simulink model "sm_car_"  (R2026b)
settings: Solver=ode23t  StopTime=100  MaxStep=0.4  AbsTol=1e-3  EnableMultiTasking=on
PreLoadFcn:
  | % Due to usability issue in Repeating Sequence block
  | warning('off','Simulink:Masking:Invalid');
  | 
  | % Eliminate unnecessary warnings in inactive variants
  | % Warnings generated only if you click through inactive variant
  | warning('off','MATLAB:nonExistentField');
  | warning('off','Simulink:Parameters:BlkParamUndefined');
PostLoadFcn:
  | set_param([bdroot '/Vehicle'],'popup_trailer','Off')
  | warning('off','sm:sli:setup:compile:LocalSolverNotSupported')
  | %sm_car_config_maneuver(bdroot,'WOT Braking');
  | sm_car_config_vehicle(bdroot,'false');
  | sm_car_config_logging(bdroot);
InitFcn:
  | sm_car_config_camera;
  | Vehicle = sm_car_vehcfg_checkConfig(Vehicle);
  | sm_car_check_tire_model(bdroot);
StartFcn:
  | tic;
StopFcn:
  | Elapsed_Sim_Time = toc;
  | % disp(['Elapsed Sim Time = ' num2str(Elapsed_Sim_Time)]);
undefined symbols (not defined in the file or in its folder): acc_theta, accel_ramp_rate, Axle1D, AxleIn, Camera, Control, Driver, Init, Maneuver, Pedal, Scene, ShaftL1, ShaftL2, ShaftR1, ShaftR2, Visual, X, xy_data_car_side, Y, Z
libraries: sm_lib x290, fl_lib x171, nesl_utility x144, simulink x60, simulink_extras x14, sdl_lib x14, SimscapeFluids_lib x7, Damper_Element x4, Tire_1x2x x4, ee_lib x3, Scene_Utilities x3, sharedTrackingLibrary x2
(part 5 of 22)

== system sm_car_/Visualization/Data for Unreal ==
  VehBus : Inport
  DrvBus : Inport  Port=2
  Bus Selector : BusSelector  OutputSignals=aSteerWheel
  Bus Selector1 : BusSelector  OutputSignals=World.x,World.y,World.z  OutputAsBus=on
  Bus Selector2 : BusSelector  OutputSignals=World.aRoll,World.aPitch,World.aYaw  OutputAsBus=on
  Bus Selector5 : BusSelector  OutputSignals=Chassis.WhlL1.n,Chassis.WhlR1.n,Chassis.WhlL2.n,Chassis.WhlR2.n
  Bus Selector6 : BusSelector  OutputSignals=Chassis.WhlL1.aCamber,Chassis.WhlR1.aCamber,Chassis.WhlL2.aCamber,Chassis.WhlR2.aCamber
  Mux : Mux
  Mux1 : Mux
  xyz : Outport  VectorParamsAs1DForOutWhenUnconnected=off
  rpy : Outport  Port=2  VectorParamsAs1DForOutWhenUnconnected=off
  ws : Outport  Port=3  VectorParamsAs1DForOutWhenUnconnected=off
  aCamber : Outport  Port=4  VectorParamsAs1DForOutWhenUnconnected=off
  aSteerWheel : Outport  Port=5  VectorParamsAs1DForOutWhenUnconnected=off
  wires:
  Bus Selector/1 -> aSteerWheel/1  "<aSteerWheel>"
  Bus Selector6/4 -> Mux1/4  "<aCamber>"
  Bus Selector6/3 -> Mux1/3  "<aCamber>"
  Bus Selector6/2 -> Mux1/2  "<aCamber>"
  Mux/1 -> ws/1  "ws"
  Bus Selector2/1 -> rpy/1  "rpy"
  Bus Selector6/1 -> Mux1/1  "<aCamber>"
  Bus Selector5/1 -> Mux/1  "<n>"
  Bus Selector5/2 -> Mux/2  "<n>"
  Bus Selector5/4 -> Mux/4  "<n>"
  DrvBus/1 -> Bus Selector/1
  VehBus/1 -> Bus Selector1/1, Bus Selector2/1, Bus Selector5/1, Bus Selector6/1
  Mux1/1 -> aCamber/1  "aCamber"
  Bus Selector1/1 -> xyz/1  "xyz"
  Bus Selector5/3 -> Mux/3  "<n>"

== system sm_car_/Visualization/Mechanics Explorer Torque Bars ==
  CtrlBus : Inport
  RL 100 Percent Tick Offset : sm_lib/Frames and Transforms/Rigid Transform  RotationMethod=None  FollAlignAxisA=+X  BaseAlignAxisA=+Y  FollAlignAxisB=+Y  BaseAlignAxisB=+Z  RotationStandardAxis=+Z  RotationAngle=0  RotationAngleUnits=deg  RotationArbitraryAxis=[0 0 1]  RotationSequenceAxes=FollowerAxes  RotationSequence=XYX  RotationSequenceAngles=[0 0 0]  RotationSequenceAnglesUnits=deg  RotationMatrix=[1 0 0;0 1 0;0 0 1]  Quaternion=[1 0 0 0]  TranslationMethod=Cartesian  TranslationCartesianOffset=[0, 0, Visual.TorqueBars.travel]  TranslationCartesianOffsetUnits=m  TranslationStandardAxis=+Z  TranslationStandardOffset=0  TranslationStandardOffsetUnits=m  TranslationROffset=0  TranslationROffsetUnits=m  TranslationThetaOffset=0  TranslationThetaOffsetUnits=deg  TranslationZOffset=0  TranslationZOffsetUnits=m
  RL Bar Base : sm_lib/Frames and Transforms/Rigid Transform  RotationMethod=None  FollAlignAxisA=+X  BaseAlignAxisA=+Y  FollAlignAxisB=+Y  BaseAlignAxisB=+Z  RotationStandardAxis=+Z  RotationAngle=0  RotationAngleUnits=deg  RotationArbitraryAxis=[0 0 1]  RotationSequenceAxes=FollowerAxes  RotationSequence=XYX  RotationSequenceAngles=[0 0 0]  RotationSequenceAnglesUnits=deg  RotationMatrix=[1 0 0;0 1 0;0 0 1]  Quaternion=[1 0 0 0]  TranslationMethod=Cartesian  TranslationCartesianOffset=Vehicle.Chassis.Body.sAxle2.Value + [Vehicle.Chassis.SuspA2.Linkage.Upright.sWheelCentre.Value(1), abs(Vehicle.Chassis.SuspA2.Linkage.Upright.sWheelCentre.Value(2)) + Visual.TorqueBars.yOffset, Vehicle.Chassis.SuspA2.Linkage.Upright.sWheelCentre.Value(3) + Visual.TorqueBars.zOffset]  TranslationCartesianOffsetUnits=m  TranslationStandardAxis=+Z  TranslationStandardOffset=0  TranslationStandardOffsetUnits=m  TranslationROffset=0  TranslationROffsetUnits=m  TranslationThetaOffset=0  TranslationThetaOffsetUnits=deg  TranslationZOffset=0  TranslationZOffsetUnits=m
  RL Clip 0 100 : Saturate  UpperLimit=1  LowerLimit=0
  RL Demand Marker : sm_lib/Body Elements/Graphic  GraphicType=Marker  MarkerShape=Cube  MarkerSize=Visual.TorqueBars.markerSize +2  GraphicVisPropType=SimpleVisualProperties  GraphicDiffuseColor=Visual.TorqueBars.fill.clr  GraphicOpacity=Visual.TorqueBars.fill.opc*torque_bar_opacity_scale  GraphicSpecularColor=[0.5 0.5 0.5 1.0]  GraphicAmbientColor=[0.15 0.15 0.15 1.0]  GraphicEmissiveColor=[0.0 0.0 0.0 1.0]  GraphicShininess=75
  RL Demand Visual Memory : Memory
  RL Demand to Position : nesl_utility/Simulink-PS Converter  PhysicalDomain=network_engine_domain  SubClassName=ps_input  LeftPortType=input  RightPortType=output  PseudoPeriodic=off  Frequencies=[]  NoiseDistribution=none  NoiseParameters=[]  Unit=m  AffineConversion=off  FilteringAndDerivatives=filter  SimscapeFilterOrder=2  InputFilterTimeConstant=Visual.TorqueBars.filterTimeConstant  UdotUserProvided=0
  RL Full Tick : sm_lib/Body Elements/Graphic  GraphicType=Marker  MarkerShape=Cube  MarkerSize=Visual.TorqueBars.markerSize  GraphicVisPropType=SimpleVisualProperties  GraphicDiffuseColor=Visual.TorqueBars.tick.clr  GraphicOpacity=Visual.TorqueBars.tick.opc*torque_bar_opacity_scale  GraphicSpecularColor=[0.5 0.5 0.5 1.0]  GraphicAmbientColor=[0.15 0.15 0.15 1.0]  GraphicEmissiveColor=[0.0 0.0 0.0 1.0]  GraphicShininess=75
  RL Percent : Gain  Gain=1/max(Vehicle.Powertrain.Power.Motor.TorqueSpd.trq.Value)
  RL Toggle : Gain  Gain=torque_bar_enable
  RL Torque Slider : sm_lib/Joints/Prismatic Joint  JointMode=Normal  CompositeWrenchDir=FollowerOnBase  CompositeWrenchFrame=BaseFrame  SenseConstraintForce=off  SenseConstraintTorque=off  SenseTotalForce=off  SenseTotalTorque=off  PositionTargetSpecify=off  PositionTargetPriority=High  PositionTargetValue=0  PositionTargetValueUnits=m  VelocityTargetSpecify=off  VelocityTargetPriority=High  VelocityTargetValue=0  VelocityTargetValueUnits=m/s  EquilibriumPosition=0  EquilibriumPositionUnits=m  SpringStiffness=0  SpringStiffnessUnits=N/m  DampingCoefficient=0  DampingCoefficientUnits=N/(m/s)  LowerLimitSpecify=off  LowerLimitBound=-1  LowerLimitBoundUnits=m  LowerLimitStiffness=1e6  LowerLimitStiffnessUnits=N/m  LowerLimitDamping=1e3  LowerLimitDampingUnits=N/(m/s)  LowerLimitTransitionRegionWidth=1e-4  LowerLimitTransitionRegionWidthUnits=m  UpperLimitSpecify=off  UpperLimitBound=1  UpperLimitBoundUnits=m  UpperLimitStiffness=1e6  UpperLimitStiffnessUnits=N/m  UpperLimitDamping=1e3  UpperLimitDampingUnits=N/(m/s)  UpperLimitTransitionRegionWidth=1e-4  UpperLimitTransitionRegionWidthUnits=m  TorqueActuationMode=ComputedTorque  MotionActuationMode=InputMotion  SensePosition=off  SenseVelocity=off  SenseAcceleration=off  SenseTorqueForce=off  SenseLowerLimitTorqueForce=off  SenseUpperLimitTorqueForce=off
  RL Travel : Gain  Gain=Visual.TorqueBars.travel
  RL Zero Tick : sm_lib/Body Elements/Graphic  GraphicType=Marker  MarkerShape=Cube  MarkerSize=Visual.TorqueBars.markerSize  GraphicVisPropType=SimpleVisualProperties  GraphicDiffuseColor=Visual.TorqueBars.rail.clr  GraphicOpacity=Visual.TorqueBars.rail.opc*torque_bar_opacity_scale  GraphicSpecularColor=[0.5 0.5 0.5 1.0]  GraphicAmbientColor=[0.15 0.15 0.15 1.0]  GraphicEmissiveColor=[0.0 0.0 0.0 1.0]  GraphicShininess=75
  RR 100 Percent Tick Offset : sm_lib/Frames and Transforms/Rigid Transform  RotationMethod=None  FollAlignAxisA=+X  BaseAlignAxisA=+Y  FollAlignAxisB=+Y  BaseAlignAxisB=+Z  RotationStandardAxis=+Z  RotationAngle=0  RotationAngleUnits=deg  RotationArbitraryAxis=[0 0 1]  RotationSequenceAxes=FollowerAxes  RotationSequence=XYX  RotationSequenceAngles=[0 0 0]  RotationSequenceAnglesUnits=deg  RotationMatrix=[1 0 0;0 1 0;0 0 1]  Quaternion=[1 0 0 0]  TranslationMethod=Cartesian  TranslationCartesianOffset=[0, 0, Visual.TorqueBars.travel]  TranslationCartesianOffsetUnits=m  TranslationStandardAxis=+Z  TranslationStandardOffset=0  TranslationStandardOffsetUnits=m  TranslationROffset=0  TranslationROffsetUnits=m  TranslationThetaOffset=0  TranslationThetaOffsetUnits=deg  TranslationZOffset=0  TranslationZOffsetUnits=m
  RR Bar Base : sm_lib/Frames and Transforms/Rigid Transform  RotationMethod=None  FollAlignAxisA=+X  BaseAlignAxisA=+Y  FollAlignAxisB=+Y  BaseAlignAxisB=+Z  RotationStandardAxis=+Z  RotationAngle=0  RotationAngleUnits=deg  RotationArbitraryAxis=[0 0 1]  RotationSequenceAxes=FollowerAxes  RotationSequence=XYX  RotationSequenceAngles=[0 0 0]  RotationSequenceAnglesUnits=deg  RotationMatrix=[1 0 0;0 1 0;0 0 1]  Quaternion=[1 0 0 0]  TranslationMethod=Cartesian  TranslationCartesianOffset=Vehicle.Chassis.Body.sAxle2.Value + [Vehicle.Chassis.SuspA2.Linkage.Upright.sWheelCentre.Value(1), -(abs(Vehicle.Chassis.SuspA2.Linkage.Upright.sWheelCentre.Value(2)) + Visual.TorqueBars.yOffset), Vehicle.Chassis.SuspA2.Linkage.Upright.sWheelCentre.Value(3) + Visual.TorqueBars.zOffset]  TranslationCartesianOffsetUnits=m  TranslationStandardAxis=+Z  TranslationStandardOffset=0  TranslationStandardOffsetUnits=m  TranslationROffset=0  TranslationROffsetUnits=m  TranslationThetaOffset=0  TranslationThetaOffsetUnits=deg  TranslationZOffset=0  TranslationZOffsetUnits=m
  RR Clip 0 100 : Saturate  UpperLimit=1  LowerLimit=0
  RR Demand Marker : sm_lib/Body Elements/Graphic  GraphicType=Marker  MarkerShape=Cube  MarkerSize=Visual.TorqueBars.markerSize +2  GraphicVisPropType=SimpleVisualProperties  GraphicDiffuseColor=Visual.TorqueBars.fill.clr  GraphicOpacity=Visual.TorqueBars.fill.opc*torque_bar_opacity_scale  GraphicSpecularColor=[0.5 0.5 0.5 1.0]  GraphicAmbientColor=[0.15 0.15 0.15 1.0]  GraphicEmissiveColor=[0.0 0.0 0.0 1.0]  GraphicShininess=75
  RR Demand Visual Memory : Memory
  RR Demand to Position : nesl_utility/Simulink-PS Converter  PhysicalDomain=network_engine_domain  SubClassName=ps_input  LeftPortType=input  RightPortType=output  PseudoPeriodic=off  Frequencies=[]  NoiseDistribution=none  NoiseParameters=[]  Unit=m  AffineConversion=off  FilteringAndDerivatives=filter  SimscapeFilterOrder=2  InputFilterTimeConstant=Visual.TorqueBars.filterTimeConstant  UdotUserProvided=0
  RR Full Tick : sm_lib/Body Elements/Graphic  GraphicType=Marker  MarkerShape=Cube  MarkerSize=Visual.TorqueBars.markerSize  GraphicVisPropType=SimpleVisualProperties  GraphicDiffuseColor=Visual.TorqueBars.tick.clr  GraphicOpacity=Visual.TorqueBars.tick.opc*torque_bar_opacity_scale  GraphicSpecularColor=[0.5 0.5 0.5 1.0]  GraphicAmbientColor=[0.15 0.15 0.15 1.0]  GraphicEmissiveColor=[0.0 0.0 0.0 1.0]  GraphicShininess=75
  RR Percent : Gain  Gain=1/max(Vehicle.Powertrain.Power.Motor.TorqueSpd.trq.Value)
  RR Toggle : Gain  Gain=torque_bar_enable
  RR Torque Slider : sm_lib/Joints/Prismatic Joint  JointMode=Normal  CompositeWrenchDir=FollowerOnBase  CompositeWrenchFrame=BaseFrame  SenseConstraintForce=off  SenseConstraintTorque=off  SenseTotalForce=off  SenseTotalTorque=off  PositionTargetSpecify=off  PositionTargetPriority=High  PositionTargetValue=0  PositionTargetValueUnits=m  VelocityTargetSpecify=off  VelocityTargetPriority=High  VelocityTargetValue=0  VelocityTargetValueUnits=m/s  EquilibriumPosition=0  EquilibriumPositionUnits=m  SpringStiffness=0  SpringStiffnessUnits=N/m  DampingCoefficient=0  DampingCoefficientUnits=N/(m/s)  LowerLimitSpecify=off  LowerLimitBound=-1  LowerLimitBoundUnits=m  LowerLimitStiffness=1e6  LowerLimitStiffnessUnits=N/m  LowerLimitDamping=1e3  LowerLimitDampingUnits=N/(m/s)  LowerLimitTransitionRegionWidth=1e-4  LowerLimitTransitionRegionWidthUnits=m  UpperLimitSpecify=off  UpperLimitBound=1  UpperLimitBoundUnits=m  UpperLimitStiffness=1e6  UpperLimitStiffnessUnits=N/m  UpperLimitDamping=1e3  UpperLimitDampingUnits=N/(m/s)  UpperLimitTransitionRegionWidth=1e-4  UpperLimitTransitionRegionWidthUnits=m  TorqueActuationMode=ComputedTorque  MotionActuationMode=InputMotion  SensePosition=off  SenseVelocity=off  SenseAcceleration=off  SenseTorqueForce=off  SenseLowerLimitTorqueForce=off  SenseUpperLimitTorqueForce=off
  RR Travel : Gain  Gain=Visual.TorqueBars.travel
  RR Zero Tick : sm_lib/Body Elements/Graphic  GraphicType=Marker  MarkerShape=Cube  MarkerSize=Visual.TorqueBars.markerSize  GraphicVisPropType=SimpleVisualProperties  GraphicDiffuseColor=Visual.TorqueBars.rail.clr  GraphicOpacity=Visual.TorqueBars.rail.opc*torque_bar_opacity_scale  GraphicSpecularColor=[0.5 0.5 0.5 1.0]  GraphicAmbientColor=[0.15 0.15 0.15 1.0]  GraphicEmissiveColor=[0.0 0.0 0.0 1.0]  GraphicShininess=75
  Rear Motor Demands : BusSelector  OutputSignals=Power.MMotorL2Demand,Power.MMotorR2Demand
  Vehicle Frame : PMIOPort  Side=Left
  wires:
  RL Travel/1 -> RL Demand to Position/1
  RL Toggle/1 -> RL Travel/1
  RR Percent/1 -> RR Clip 0 100/1
  RR Toggle/1 -> RR Travel/1
  RL Clip 0 100/1 -> RL Toggle/1
  RR Travel/1 -> RR Demand to Position/1
  CtrlBus/1 -> Rear Motor Demands/1
  RL Percent/1 -> RL Clip 0 100/1
  RR Clip 0 100/1 -> RR Toggle/1
  Rear Motor Demands/1 -> RL Demand Visual Memory/1  "<MMotorL2Demand>"
  RL Demand Visual Memory/1 -> RL Percent/1  "MMotorL2Demand"
  Rear Motor Demands/2 -> RR Demand Visual Memory/1  "<MMotorR2Demand>"
  RR Demand Visual Memory/1 -> RR Percent/1  "MMotorR2Demand"
  connections:
  RR 100 Percent Tick Offset/RConn1 -- RR Full Tick/RConn1
  RR Torque Slider/RConn1 -- RR Demand Marker/RConn1
  RR Bar Base/RConn1 -- RR 100 Percent Tick Offset/LConn1 -- RR Torque Slider/LConn1 -- RR Zero Tick/RConn1
  RL Demand to Position/RConn1 -- RL Torque Slider/LConn2
  Vehicle Frame/RConn1 -- RR Bar Base/LConn1 -- RL Bar Base/LConn1
  RL Torque Slider/RConn1 -- RL Demand Marker/RConn1
  RL 100 Percent Tick Offset/RConn1 -- RL Full Tick/RConn1
  RL Zero Tick/RConn1 -- RL Torque Slider/LConn1 -- RL Bar Base/RConn1 -- RL 100 Percent Tick Offset/LConn1
  RR Demand to Position/RConn1 -- RR Torque Slider/LConn2

== system sm_car_/Visualization/Unreal ==
  "xyz " : Inport
  "rpy " : Inport  Port=2
  "ws " : Inport  Port=3
  "aCamber " : Inport  Port=4
  "aSteerWheel " : Inport  Port=5
  Animation Off : Subsystem  VariantControl=Off

== system sm_car_/World/Mechanism Configuration ==
  Constant Gravity : Subsystem  VariantControl=ConstantGravity
  Variable GravityXY : Subsystem  VariantControl=VariableGravityXY
  C : PMIOPort  Side=Right

== system sm_car_/World/Scene ==
  CRG Balkans : sm_car_scene_crg_balkans/CRG Balkans  VariantControl=CRG_Balkans  geometry=Scene.CRG_Balkans.Geometry
  CRG Balkans End : sm_car_scene_crg_balkans_end/CRG Balkans End  VariantControl=CRG_Balkans_End  geometry=Scene.CRG_Balkans_End.Geometry
  CRG Balkans End F : sm_car_scene_crg_balkans_end_f/CRG Balkans End F  VariantControl=CRG_Balkans_End_F  geometry=Scene.CRG_Balkans_End_F.Geometry
  CRG Balkans F : sm_car_scene_crg_balkans_f/CRG Balkans F  VariantControl=CRG_Balkans_F  geometry=Scene.CRG_Balkans_F.Geometry
  CRG Dej Wide : sm_car_scene_crg_dej_wide/CRG Dej Wide  VariantControl=CRG_Dej_Wide  geometry=Scene.CRG_Dej_Wide.Geometry
  CRG Dej Wide F : sm_car_scene_crg_dej_wide_f/CRG Dej Wide F  VariantControl=CRG_Dej_Wide_F  geometry=Scene.CRG_Dej_Wide_F.Geometry
  CRG Germania : sm_car_scene_crg_germania/CRG Germania  VariantControl=CRG_Germania  geometry=Scene.CRG_Germania.Geometry
  CRG Germania F : sm_car_scene_crg_germania_f/CRG Germania F  VariantControl=CRG_Germania_F  geometry=Scene.CRG_Germania_F.Geometry
  CRG Hockenheim : Subsystem  VariantControl=CRG_Hockenheim  mask{geometry=Scene.CRG_Hockenheim.Geometry}
      mask prompts: geometry "Geometry (structure)"
  CRG Hockenheim F : Subsystem  VariantControl=CRG_Hockenheim_F  mask{geometry=Scene.CRG_Hockenheim_F.Geometry}
      mask prompts: geometry "Geometry (structure)"
  Double Lane Change : Subsystem  VariantControl=Double_Lane_Change  mask{road=Scene.Double_Lane_Change.Road, dashes=Scene.Double_Lane_Change.Dashes, cones=Scene.Double_Lane_Change.Cones}
      mask prompts: road "Road (structure)"; dashes "Dashes (structure)"; cones "Cones (structure)"
  Plane Grid : Subsystem  VariantControl=Plane_Grid  mask{plane=Scene.Plane_Grid.Plane, grid=Scene.Plane_Grid.Grid}
      mask prompts: plane "Ground Plane (structure)"; grid "Grid (structure)"
  Skidpad : Subsystem  VariantControl=Skidpad  mask{circ_in=Scene.Skidpad.Circle_Inner, circ_out=Scene.Skidpad.Circle_Outer, plane=Scene.Skidpad.Plane}
      mask prompts: circ_in "Circle Inner (structure)"; circ_out "Circle Outer (structure)"; plane "Plane (structure)"
  Slalom : sm_car_scene_slalom/Slalom  VariantControl=Slalom  road=Scene.Slalom.Road  dashes=Scene.Slalom.Dashes  cones=Scene.Slalom.Cones  vehTraj=Maneuver.Trajectory
  W : PMIOPort  Side=Left
  Obs : Outport  VectorParamsAs1DForOutWhenUnconnected=off

== system sm_car_/Camera Frames/Dolly Camera/Off ==
  W : PMIOPort  Side=Left
  R : PMIOPort  Port=2  Side=Right
  connections:
  R/RConn1 -- W/RConn1

== system sm_car_/Controller/Default/Brake Control ==
  "rBrakePedal " : Inport
  "VehBus " : Inport  Port=2
  Pedal : Subsystem  VariantControl=Pedal
  " Brakes" : Outport  VectorParamsAs1DForOutWhenUnconnected=off

== system sm_car_/Controller/Default/Driveline Control ==
  Bus Creator : BusCreator  Inputs=1
  Constant : Constant  Value=0
  Driveline : Outport  VectorParamsAs1DForOutWhenUnconnected=off
  wires:
  Bus Creator/1 -> Driveline/1  "Driveline"
  Constant/1 -> Bus Creator/1  "placeholder"

== system sm_car_/Controller/Default/Power Control ==
  note: For 4 Motor Powertrain only
  note: For 2 Motor Powertrain only
  rAccelPedal : Inport
  VehBus : Inport  Port=2
  StatesEst : Inport  Port=3
  1-D Lookup Table : Lookup_n-D  NumberOfTableDimensions=1  BreakpointsForDimension1=[0;400;4600]  Table=[0;3;8]  InternalRulePriority=Speed  RndMeth=Simplest
  1-D Lookup Table1 : Lookup_n-D  NumberOfTableDimensions=1  BreakpointsForDimension1=[-1;-0.20000000000000001;-0.10000000000000001;0;0.10000000000000001;0.20000000000000001;1]  Table=[0;0;1;1;1;0;0]  InternalRulePriority=Speed  RndMeth=Simplest
  1-D Lookup Table2 : Lookup_n-D  NumberOfTableDimensions=1  BreakpointsForDimension1=[0;400;4600]  Table=[0;3;8]  InternalRulePriority=Speed  RndMeth=Simplest
  Add : Sum
  Add1 : Sum
  Bus Creator : BusCreator  Inputs=7
  Bus Selector : BusSelector  OutputSignals=Power.MotorL2.w,Power.MotorR2.w
  Constant : Constant  Value=trq_ratio_front
  Constant1 : Constant  Value=0
  Constant2 : Constant
  Gain : Gain  Gain=max(Vehicle.Powertrain.Power.Motor.TorqueSpd.trq.Value)
  Gain1 : Gain  Gain=-1
  Gain2 : Gain  Gain=-1
  Gain3 : Gain  Gain=0.5
  Gain4 : Gain  Gain=0.5
  Product{,1..3} (4 alike) : Product
  Rate Limiter : RateLimiter  RisingSlewLimit=trq_rate_up  FallingSlewLimit=trq_rate_down  SampleTimeMode=inherited
  Terminator1 : Terminator
  Power : Outport  VectorParamsAs1DForOutWhenUnconnected=off
  wires:
  Bus Creator/1 -> Power/1  "Power"
  Product1/1 -> Add1/1, Add/1, Bus Creator/4  "MMotorA2Demand"
  Gain/1 -> 1-D Lookup Table1/1, Rate Limiter/1
  Product/1 -> Gain4/1, Gain3/1, Bus Creator/1  "MMotorA1Demand"
  rAccelPedal/1 -> Gain/1
  VehBus/1 -> Bus Selector/1
  Constant1/1 -> Bus Creator/7  "MRegenBrakeLimit"
  Rate Limiter/1 -> Product1/1, Product/2
  Constant/1 -> Product/1
  Constant2/1 -> Product1/2
  Add/1 -> Bus Creator/5  "MMotorL2Demand"
  Add1/1 -> Bus Creator/6  "MMotorR2Demand"
  Gain3/1 -> Bus Creator/2  "MMotorL1Demand"
  Gain4/1 -> Bus Creator/3  "MMotorR1Demand"
  StatesEst/1 -> Terminator1/1
  Bus Selector/1 -> 1-D Lookup Table/1  "<w>"
  Bus Selector/2 -> 1-D Lookup Table2/1  "<w>"
  1-D Lookup Table/1 -> Gain1/1
  1-D Lookup Table1/1 -> Product3/1, Product2/1
  1-D Lookup Table2/1 -> Gain2/1
  Product2/1 -> Add/2
  Product3/1 -> Add1/2
  Gain1/1 -> Product2/2
  Gain2/1 -> Product3/2

== system sm_car_/Controller/Default/Spring Damper ==
  Bus Creator : BusCreator  Inputs=4
  Bus Creator1 : BusCreator  Inputs=4
  Constant : Constant  Value=[0 0 0 0]
  Constant1 : Constant  Value=[0 0 0 0]
  Demux : Demux
  Demux1 : Demux
  Damper : Outport  VectorParamsAs1DForOutWhenUnconnected=off
  Spring : Outport  Port=2  VectorParamsAs1DForOutWhenUnconnected=off
  wires:
  Constant/1 -> Demux/1
  Demux/3 -> Bus Creator/3  "L2"
  Demux/4 -> Bus Creator/4  "R2"
  Demux/1 -> Bus Creator/1  "L1"
  Demux/2 -> Bus Creator/2  "R1"
  Demux1/2 -> Bus Creator1/2  "R1"
  Demux1/1 -> Bus Creator1/1  "L1"
  Demux1/4 -> Bus Creator1/4  "R2"
  Demux1/3 -> Bus Creator1/3  "L2"
  Constant1/1 -> Demux1/1
  Bus Creator1/1 -> Damper/1  "Damper"
  Bus Creator/1 -> Spring/1  "Spring"

== system sm_car_/Controller/Default/State Estimation ==
  aSteerWheel : Inport
  VehBus : Inport  Port=2
  Bus Creator : BusCreator  Inputs=5
  Bus Selector : BusSelector  OutputSignals=World.vx,World.vy,World.vz,Chassis.Body.CG.nYaw,Chassis.Body.CG.gx,Chassis.Body.CG.gy,Chassis.SuspA1.LinkageL.Upright.Upright.w,Chassis.SuspA1.LinkageR.Upright.Upright.w,Chassis.SuspA2.LinkageL.Upright.Upright.w,Chassis.SuspA2.LinkageR.Upright.Upright.w
  Data Type Conversion : DataTypeConversion  OutDataTypeStr=double  SaturateOnIntegerOverflow=off  RndMeth=Floor
  Data Type Conversion1 : DataTypeConversion  OutDataTypeStr=double  SaturateOnIntegerOverflow=off  RndMeth=Floor
  Demux : Demux  Outputs=5
  Rate Transition1 : RateTransition  Deterministic=off  OutPortSampleTime=0.003
  Rate Transition2 : RateTransition  Deterministic=off  OutPortSampleTime=0.003
  Rate Transition4 : RateTransition  Deterministic=off
  Sensor Noise Simulation : Subsystem
  UKF : Subsystem
  StateEst : Outport
  Out Bus Element : Outport  Port=2  PortName=Meas  Element=Meas
  Out Bus Element1 : Outport  Port=2  PortName=Meas  Element=Input
  Out Bus Element2 : Outport  Port=2  PortName=Meas  Element=State
  wires:
  VehBus/1 -> Bus Selector/1
  Bus Selector/1 -> Sensor Noise Simulation/1(<vx>)  "<vx>"
  Bus Selector/2 -> Sensor Noise Simulation/2(<vy>)  "<vy>"
  Bus Selector/4 -> Sensor Noise Simulation/4(<nYaw>)  "<nYaw>"
  Bus Selector/5 -> Sensor Noise Simulation/5(<gx>)  "<gx>"
  Bus Selector/6 -> Sensor Noise Simulation/6(<gy>)  "<gy>"
  Bus Selector/7 -> Sensor Noise Simulation/7(<w_fl>)  "<w>"
  Bus Selector/8 -> Sensor Noise Simulation/8(<w_fr>)  "<w>"
  Bus Selector/9 -> Sensor Noise Simulation/9(<w_rl>)  "<w>"
  Bus Selector/10 -> Sensor Noise Simulation/10(<w_rr>)  "<w>"
  aSteerWheel/1 -> Sensor Noise Simulation/11(delta)  "delta"
  Sensor Noise Simulation/2(Meas) -> Rate Transition2/1, Out Bus Element/1  "Measument"
  Sensor Noise Simulation/1(Inputs) -> Data Type Conversion1/1, Rate Transition1/1  "Input"
  Data Type Conversion/1 -> Demux/1
  Bus Creator/1 -> Out Bus Element2/1, StateEst/1  "UKF"
  Demux/1 -> Bus Creator/1  "v_x"
  Demux/2 -> Bus Creator/2  "v_y"
  Demux/3 -> Bus Creator/3  "phi_dot"
  Demux/4 -> Bus Creator/4  "a_x"
  Demux/5 -> Bus Creator/5  "a_y"
  Rate Transition1/1 -> UKF/1(StateTransitionFcnInputs)
  Rate Transition2/1 -> UKF/2(y1)
  UKF/1(xhat) -> Data Type Conversion/1
  Data Type Conversion1/1 -> Rate Transition4/1
  Rate Transition4/1 -> Out Bus Element1/1
  Bus Selector/3 -> Sensor Noise Simulation/3(<vz>)  "<vz>"

== system sm_car_/Controller/Default/Susp ==
  aSteerWheel : Inport
  vx : Inport  Port=2
  1-D Lookup Table : Lookup_n-D  NumberOfTableDimensions=1  BreakpointsForDimension1=Steer.Gain.vVehicle.Value  Table=Steer.Gain.n.Value  InterpMethod=Linear Lagrange  InternalRulePriority=Speed  RndMeth=Simplest
  Bus Creator{1..4} (4 alike) : BusCreator  Inputs=1
  Gain : Gain  Gain=3.6
  Product : Product
  Saturation : Saturate  UpperLimit=Steer.Limits.aUpper.Value  LowerLimit=Steer.Limits.aLower.Value  LinearizeAsGain=off  ZeroCross=off
  Transfer Fcn (with initial states) : simulink_extras/Additional Linear/Transfer Fcn (with initial states)  N=[1]  D="[1/Steer.fActuatorCutoff.Value  1]"  X0=-1
  SuspA1 : Outport  VectorParamsAs1DForOutWhenUnconnected=off
  SuspA2 : Outport  Port=2  VectorParamsAs1DForOutWhenUnconnected=off
  wires:
  Bus Creator4/1 -> Bus Creator1/1  "Steer"
  Bus Creator2/1 -> Bus Creator3/1  "Steer"
  Bus Creator3/1 -> SuspA2/1  "SuspA2"
  Bus Creator1/1 -> SuspA1/1  "SuspA1"
  aSteerWheel/1 -> Product/1, Bus Creator4/1  "aSteerWheel"
  Saturation/1 -> Bus Creator2/1  "aSteerWheel"
  vx/1 -> Gain/1
  Transfer Fcn (with initial states)/1 -> Product/2
  Product/1 -> Saturation/1
  Gain/1 -> 1-D Lookup Table/1
  1-D Lookup Table/1 -> Transfer Fcn (with initial states)/1

== system sm_car_/Controller/FeedF_Ctrl/Brake Control ==
  "rBrakePedal " : Inport
  "VehBus " : Inport  Port=2
  Pedal : Subsystem  VariantControl=Pedal
  " Brakes" : Outport  VectorParamsAs1DForOutWhenUnconnected=off

== system sm_car_/Controller/FeedF_Ctrl/Driveline Control ==
  Bus Creator : BusCreator  Inputs=1
  Constant : Constant  Value=0
  Driveline : Outport  VectorParamsAs1DForOutWhenUnconnected=off
  wires:
  Constant/1 -> Bus Creator/1  "placeholder"
  Bus Creator/1 -> Driveline/1  "Driveline"

== system sm_car_/Controller/FeedF_Ctrl/Power Control ==
  rAccelPedal : Inport
  VehBus : Inport  Port=2
  aSteerWheel : Inport  Port=3
  Bias : Bias  Bias=512  SaturateOnIntegerOverflow=off
  Bus Creator : BusCreator  Inputs=2
  Bus Selector : BusSelector  OutputSignals=Power.MotorL2.w,Power.MotorR2.w
  Gain : Gain  Gain=max(Control.MotorTrq)
  Gain1 : Gain  Gain=max(Control.MotorTrq)
  Gain3 : Gain  Gain=511/154
  Radians to Degrees : simulink_extras/Transformations/Radians to Degrees
  Subsystem Reference : Subsystem  ReferencedSubsystem=FeedForward  rwheel=Control.WheelRad  L=Control.Wheelbase  StrWhlRatio=Control.StrWheelRatio  Izz=Control.Izz  tr=Control.RearTrack  Gr=Control.GearRatio  MotorT=Control.MotorTrq  MotorW=Control.MotorW  Tf=0.005  Tmax=max(Control.MotorTrq)  Ku=Control.UndersteerGradient
  Power : Outport  VectorParamsAs1DForOutWhenUnconnected=off
  wires:
  Bias/1 -> Subsystem Reference/1
  Gain3/1 -> Bias/1
  Radians to Degrees/1 -> Gain3/1
  Gain1/1 -> Bus Creator/2  "MMotorR2Demand"
  Gain/1 -> Bus Creator/1  "MMotorL2Demand"
  Subsystem Reference/2 -> Gain1/1  "MMotorR2Demand"
  Subsystem Reference/1 -> Gain/1  "MMotorL2Demand"
  Bus Creator/1 -> Power/1
  rAccelPedal/1 -> Subsystem Reference/4  "Throttle[~]"
  aSteerWheel/1 -> Radians to Degrees/1  "Throttle[~]"
  VehBus/1 -> Bus Selector/1
  Bus Selector/1 -> Subsystem Reference/2  "<w>"
  Bus Selector/2 -> Subsystem Reference/3  "<w>"

== system sm_car_/Controller/FeedF_Ctrl/Spring Damper ==
  Bus Creator : BusCreator  Inputs=4
  Bus Creator1 : BusCreator  Inputs=4
  Constant : Constant  Value=[0 0 0 0]
  Constant1 : Constant  Value=[0 0 0 0]
  Demux : Demux
  Demux1 : Demux
  Damper : Outport  VectorParamsAs1DForOutWhenUnconnected=off
  Spring : Outport  Port=2  VectorParamsAs1DForOutWhenUnconnected=off
  wires:
  Bus Creator/1 -> Spring/1  "Spring"
  Bus Creator1/1 -> Damper/1  "Damper"
  Constant1/1 -> Demux1/1
  Demux1/3 -> Bus Creator1/3  "L2"
  Demux1/4 -> Bus Creator1/4  "R2"
  Demux1/1 -> Bus Creator1/1  "L1"
  Demux1/2 -> Bus Creator1/2  "R1"
  Demux/2 -> Bus Creator/2  "R1"
  Demux/1 -> Bus Creator/1  "L1"
  Demux/4 -> Bus Creator/4  "R2"
  Demux/3 -> Bus Creator/3  "L2"
  Constant/1 -> Demux/1

== system sm_car_/Controller/FeedF_Ctrl/Susp ==
  aSteerWheel : Inport
  vx : Inport  Port=2
  1-D Lookup Table : Lookup_n-D  NumberOfTableDimensions=1  BreakpointsForDimension1=Steer.Gain.vVehicle.Value  Table=Steer.Gain.n.Value  InterpMethod=Linear Lagrange  InternalRulePriority=Speed  RndMeth=Simplest
  Bus Creator{1..4} (4 alike) : BusCreator  Inputs=1
  Gain : Gain  Gain=3.6
  Product : Product
  Saturation : Saturate  UpperLimit=Steer.Limits.aUpper.Value  LowerLimit=Steer.Limits.aLower.Value  LinearizeAsGain=off  ZeroCross=off
  Transfer Fcn (with initial states) : simulink_extras/Additional Linear/Transfer Fcn (with initial states)  N=[1]  D="[1/Steer.fActuatorCutoff.Value  1]"  X0=-1
  SuspA1 : Outport  VectorParamsAs1DForOutWhenUnconnected=off
  SuspA2 : Outport  Port=2  VectorParamsAs1DForOutWhenUnconnected=off
  wires:
  1-D Lookup Table/1 -> Transfer Fcn (with initial states)/1
  Gain/1 -> 1-D Lookup Table/1
  Product/1 -> Saturation/1
  Transfer Fcn (with initial states)/1 -> Product/2
  vx/1 -> Gain/1
  Saturation/1 -> Bus Creator2/1  "aSteerWheel"
  aSteerWheel/1 -> Bus Creator4/1, Product/1  "aSteerWheel"
  Bus Creator1/1 -> SuspA1/1  "SuspA1"
  Bus Creator3/1 -> SuspA2/1  "SuspA2"
  Bus Creator2/1 -> Bus Creator3/1  "Steer"
  Bus Creator4/1 -> Bus Creator1/1  "Steer"

== system sm_car_/Controller/NoIMU/Brake Control ==
  "rBrakePedal " : Inport
  "VehBus " : Inport  Port=2
  Pedal : Subsystem  VariantControl=Pedal
  " Brakes" : Outport  VectorParamsAs1DForOutWhenUnconnected=off

== system sm_car_/Controller/NoIMU/Driveline Control ==
  Bus Creator : BusCreator  Inputs=1
  Constant : Constant  Value=0
  Driveline : Outport  VectorParamsAs1DForOutWhenUnconnected=off
  wires:
  Constant/1 -> Bus Creator/1  "placeholder"
  Bus Creator/1 -> Driveline/1  "Driveline"

== system sm_car_/Controller/NoIMU/Power Control ==
  rAccelPedal : Inport
  VehBus : Inport  Port=2
  Add1 : Sum
  Bus Creator : BusCreator  Inputs=2
  Bus Creator2 : BusCreator  Inputs=2
  Bus Selector : BusSelector  OutputSignals=Power.Battery.v,Power.MotorL2.i,Power.MotorR2.i
  Constant : Constant
  Current-Torque : Subsystem
  Delay : Delay  DelayLength=1  InputProcessing=Columns as channels (frame based)
  Fuzzy Logic Controller : fuzblock/Fuzzy Logic  Controller  FIS=fis  OutputSampleNumber=101  DataType=double  UseLookupTable=off  NumBreakpoints=10  FuzzifiedInputs=off  RuleFiringStrengths=off  RuleOutputs=off  AggregatedOutputs=off  SimulateUsing=Interpreted execution  OutOfRangeInputValueMessage=warning  NoRuleFiredMessage=warning  EmptyOutputFuzzySetMessage=warning
  Product : Product
  Product1 : Product
  Product2 : Product  Inputs=3
  Saturation : Saturate  UpperLimit=1  LowerLimit=0
  Slip Control : Subsystem  Commented=on
  Subtract : Sum  Inputs=+-
  Sum : Sum  Inputs=|+-
  Tmax : Gain  Gain=1/Tmax/2
  max torque : Constant  Value=Tmax
  Power : Outport  VectorParamsAs1DForOutWhenUnconnected=off
  wires:
  VehBus/1 -> Slip Control/1(VehBus), Bus Selector/1
  Bus Creator/1 -> Power/1  "Power"
  rAccelPedal/1 -> Sum/1, Product2/1  "Throttle[~]"
  Bus Selector/1 -> Current-Torque/1(V)  "<v>"
  Bus Selector/2 -> Current-Torque/2(Il)  "<i>"
  Bus Selector/3 -> Current-Torque/3(Ir)  "<i>"
  Fuzzy Logic Controller/1 -> Add1/2
  Current-Torque/1(Out1) -> Tmax/1  "Treal[Nm]"
  Bus Creator2/1 -> ?
  Product2/1 -> Product/1, Product1/1  "MDemand[Nm]"
  Tmax/1 -> Saturation/1
  Saturation/1 -> Sum/2  "Treal[%]"
  max torque/1 -> Product2/3
  Add1/1 -> Product2/2
  Sum/1 -> Delay/1, Subtract/1, Bus Creator2/1
  Delay/1 -> Subtract/2
  Subtract/1 -> Bus Creator2/2
  Constant/1 -> Add1/1
  Product/1 -> Bus Creator/2  "MMotorR2Demand"
  Product1/1 -> Bus Creator/1  "MMotorL2Demand"
  Slip Control/1(Out1) -> Product1/2
  Slip Control/2(Out2) -> Product/2

== system sm_car_/Controller/NoIMU/Spring Damper ==
  Bus Creator : BusCreator  Inputs=4
  Bus Creator1 : BusCreator  Inputs=4
  Constant : Constant  Value=[0 0 0 0]
  Constant1 : Constant  Value=[0 0 0 0]
  Demux : Demux
  Demux1 : Demux
  Damper : Outport  VectorParamsAs1DForOutWhenUnconnected=off
  Spring : Outport  Port=2  VectorParamsAs1DForOutWhenUnconnected=off
  wires:
  Bus Creator/1 -> Spring/1  "Spring"
  Bus Creator1/1 -> Damper/1  "Damper"
  Constant1/1 -> Demux1/1
  Demux1/3 -> Bus Creator1/3  "L2"
  Demux1/4 -> Bus Creator1/4  "R2"
  Demux1/1 -> Bus Creator1/1  "L1"
  Demux1/2 -> Bus Creator1/2  "R1"
  Demux/2 -> Bus Creator/2  "R1"
  Demux/1 -> Bus Creator/1  "L1"
  Demux/4 -> Bus Creator/4  "R2"
  Demux/3 -> Bus Creator/3  "L2"
  Constant/1 -> Demux/1

== system sm_car_/Controller/NoIMU/Susp ==
  aSteerWheel : Inport
  vx : Inport  Port=2
  1-D Lookup Table : Lookup_n-D  NumberOfTableDimensions=1  BreakpointsForDimension1=Steer.Gain.vVehicle.Value  Table=Steer.Gain.n.Value  InterpMethod=Linear Lagrange  InternalRulePriority=Speed  RndMeth=Simplest
  Bus Creator{1..4} (4 alike) : BusCreator  Inputs=1
  Gain : Gain  Gain=3.6
  Product : Product
  Saturation : Saturate  UpperLimit=Steer.Limits.aUpper.Value  LowerLimit=Steer.Limits.aLower.Value  LinearizeAsGain=off  ZeroCross=off
  Transfer Fcn (with initial states) : simulink_extras/Additional Linear/Transfer Fcn (with initial states)  N=[1]  D="[1/Steer.fActuatorCutoff.Value  1]"  X0=-1
  SuspA1 : Outport  VectorParamsAs1DForOutWhenUnconnected=off
  SuspA2 : Outport  Port=2  VectorParamsAs1DForOutWhenUnconnected=off
  wires:
  1-D Lookup Table/1 -> Transfer Fcn (with initial states)/1
  Gain/1 -> 1-D Lookup Table/1
  Product/1 -> Saturation/1
  Transfer Fcn (with initial states)/1 -> Product/2
  vx/1 -> Gain/1
  Saturation/1 -> Bus Creator2/1  "aSteerWheel"
  aSteerWheel/1 -> Bus Creator4/1, Product/1  "aSteerWheel"
  Bus Creator1/1 -> SuspA1/1  "SuspA1"
  Bus Creator3/1 -> SuspA2/1  "SuspA2"
  Bus Creator2/1 -> Bus Creator3/1  "Steer"
  Bus Creator4/1 -> Bus Creator1/1  "Steer"

== system sm_car_/Controller/Slip_Ctrl/Brake Control ==
  "rBrakePedal " : Inport
  "VehBus " : Inport  Port=2
  Pedal : Subsystem  VariantControl=Pedal
  " Brakes" : Outport  VectorParamsAs1DForOutWhenUnconnected=off

== system sm_car_/Controller/Slip_Ctrl/Driveline Control ==
  Bus Creator : BusCreator  Inputs=1
  Constant : Constant  Value=0
  Driveline : Outport  VectorParamsAs1DForOutWhenUnconnected=off
  wires:
  Constant/1 -> Bus Creator/1  "placeholder"
  Bus Creator/1 -> Driveline/1  "Driveline"

== system sm_car_/Controller/Slip_Ctrl/Power Control ==
  rAccelPedal : Inport
  VehBus : Inport  Port=2
  Bus Creator : BusCreator  Inputs=2
  Bus Selector : BusSelector  OutputSignals=Chassis.Body.CG.vx,Chassis.SuspA2.LinkageL.Upright.Upright.w,Chassis.SuspA2.LinkageR.Upright.Upright.w,Chassis.Body.CG.gx,Chassis.Body.CG.gy,Chassis.Body.CG.nYaw
  Gain : Gain  Gain=max(Control.MotorTrq)
  Gain1 : Gain  Gain=max(Control.MotorTrq)
  Slip Control : Subsystem  TreatAsAtomicUnit=on  ReferencedSubsystem=Slip_Control  Gr=Control.GearRatio  MotorT=Control.MotorTrq  MotorW=Control.MotorW  rwheel=Control.WheelRad  tr=Control.RearTrack  a=Control.FrontTrackToCG  a_cop=Control.FrontTrackToCoP  Af=Control.FrontalArea  P=90  I=105  N=100  D=1.2  vx_th=Control.ActivationVelocity  cd=Control.LiftCoef  g=Control.GravitationAcc  h_CG=Control.CGHeight  L=Control.Wheelbase  m=Control.Mass  ro=Control.AirDensity  Tmax=max(Control.MotorTrq)  Load_Ref=Control.LoadRef  Slip_Ref=Control.SlipRef
  Power : Outport  VectorParamsAs1DForOutWhenUnconnected=off
  wires:
  Slip Control/2 -> Gain1/1  "MMotorR2Demand"
  Slip Control/1 -> Gain/1  "MMotorL2Demand"
  Bus Creator/1 -> Power/1
  Bus Selector/6 -> Slip Control/6  "<nYaw>"
  Bus Selector/4 -> Slip Control/4  "<gx>"
  Bus Selector/5 -> Slip Control/5  "<gy>"
  Bus Selector/3 -> Slip Control/3  "<w>"
  Bus Selector/1 -> Slip Control/1  "<vx>"
  rAccelPedal/1 -> Slip Control/7  "Throttle[~]"
  VehBus/1 -> Bus Selector/1
  Bus Selector/2 -> Slip Control/2  "<w>"
  Gain/1 -> Bus Creator/1  "MMotorL2Demand"
  Gain1/1 -> Bus Creator/2  "MMotorR2Demand"

== system sm_car_/Controller/Slip_Ctrl/Spring Damper ==
  Bus Creator : BusCreator  Inputs=4
  Bus Creator1 : BusCreator  Inputs=4
  Constant : Constant  Value=[0 0 0 0]
  Constant1 : Constant  Value=[0 0 0 0]
  Demux : Demux
  Demux1 : Demux
  Damper : Outport  VectorParamsAs1DForOutWhenUnconnected=off
  Spring : Outport  Port=2  VectorParamsAs1DForOutWhenUnconnected=off
  wires:
  Bus Creator/1 -> Spring/1  "Spring"
  Bus Creator1/1 -> Damper/1  "Damper"
  Constant1/1 -> Demux1/1
  Demux1/3 -> Bus Creator1/3  "L2"
  Demux1/4 -> Bus Creator1/4  "R2"
  Demux1/1 -> Bus Creator1/1  "L1"
  Demux1/2 -> Bus Creator1/2  "R1"
  Demux/2 -> Bus Creator/2  "R1"
  Demux/1 -> Bus Creator/1  "L1"
  Demux/4 -> Bus Creator/4  "R2"
  Demux/3 -> Bus Creator/3  "L2"
  Constant/1 -> Demux/1

== system sm_car_/Controller/Slip_Ctrl/Susp ==
  aSteerWheel : Inport
  vx : Inport  Port=2
  1-D Lookup Table : Lookup_n-D  NumberOfTableDimensions=1  BreakpointsForDimension1=Steer.Gain.vVehicle.Value  Table=Steer.Gain.n.Value  InterpMethod=Linear Lagrange  InternalRulePriority=Speed  RndMeth=Simplest
  Bus Creator{1..4} (4 alike) : BusCreator  Inputs=1
  Gain : Gain  Gain=3.6
  Product : Product
  Saturation : Saturate  UpperLimit=Steer.Limits.aUpper.Value  LowerLimit=Steer.Limits.aLower.Value  LinearizeAsGain=off  ZeroCross=off
  Transfer Fcn (with initial states) : simulink_extras/Additional Linear/Transfer Fcn (with initial states)  N=[1]  D="[1/Steer.fActuatorCutoff.Value  1]"  X0=-1
  SuspA1 : Outport  VectorParamsAs1DForOutWhenUnconnected=off
  SuspA2 : Outport  Port=2  VectorParamsAs1DForOutWhenUnconnected=off
  wires:
  1-D Lookup Table/1 -> Transfer Fcn (with initial states)/1
  Gain/1 -> 1-D Lookup Table/1
  Product/1 -> Saturation/1
  Transfer Fcn (with initial states)/1 -> Product/2
  vx/1 -> Gain/1
  Saturation/1 -> Bus Creator2/1  "aSteerWheel"
  aSteerWheel/1 -> Bus Creator4/1, Product/1  "aSteerWheel"
  Bus Creator1/1 -> SuspA1/1  "SuspA1"
  Bus Creator3/1 -> SuspA2/1  "SuspA2"
  Bus Creator2/1 -> Bus Creator3/1  "Steer"
  Bus Creator4/1 -> Bus Creator1/1  "Steer"

== system sm_car_/Controller/Slip_Ctrl_V2/Brake Control ==
  "rBrakePedal " : Inport
  "VehBus " : Inport  Port=2
  Pedal : Subsystem  VariantControl=Pedal
  " Brakes" : Outport  VectorParamsAs1DForOutWhenUnconnected=off

== system sm_car_/Controller/Slip_Ctrl_V2/Driveline Control ==
  Bus Creator : BusCreator  Inputs=1
  Constant : Constant  Value=0
  Driveline : Outport  VectorParamsAs1DForOutWhenUnconnected=off
  wires:
  Bus Creator/1 -> Driveline/1  "Driveline"
  Constant/1 -> Bus Creator/1  "placeholder"

== system sm_car_/Controller/Slip_Ctrl_V2/Power Control ==
  rAccelPedal : Inport
  VehBus : Inport  Port=2
  Bus Creator : BusCreator  Inputs=2
  Bus Selector : BusSelector  OutputSignals=Chassis.Body.CG.vx,Chassis.SuspA2.LinkageL.Upright.Upright.w,Chassis.SuspA2.LinkageR.Upright.Upright.w,Chassis.Body.CG.gx,Chassis.Body.CG.gy,Chassis.Body.CG.nYaw
  Gain : Gain  Gain=max(Control.MotorTrq)
  Gain1 : Gain  Gain=max(Control.MotorTrq)
  Slip Control : Subsystem  TreatAsAtomicUnit=on  ReferencedSubsystem=Slip_Control  Gr=Control.GearRatio  MotorT=Control.MotorTrq  MotorW=Control.MotorW  rwheel=Control.WheelRad  tr=Control.RearTrack  a=Control.FrontTrackToCG  a_cop=Control.FrontTrackToCoP  Af=Control.FrontalArea  P=90  I=0  N=100  D=0.8  vx_th=Control.ActivationVelocity  cd=Control.LiftCoef  g=Control.GravitationAcc  h_CG=Control.CGHeight  L=Control.Wheelbase  m=Control.Mass  ro=Control.AirDensity  Tmax=max(Control.MotorTrq)  Load_Ref=Control.LoadRef  Slip_Ref=Control.SlipRef
  Power : Outport  VectorParamsAs1DForOutWhenUnconnected=off
  wires:
  VehBus/1 -> Bus Selector/1
  Bus Creator/1 -> Power/1
  Gain/1 -> Bus Creator/1  "MMotorL2Demand"
  Gain1/1 -> Bus Creator/2  "MMotorR2Demand"
  Bus Selector/1 -> Slip Control/1  "<vx>"
  Bus Selector/2 -> Slip Control/2  "<w>"
  Bus Selector/3 -> Slip Control/3  "<w>"
  rAccelPedal/1 -> Slip Control/7  "Throttle[~]"
  Slip Control/1 -> Gain/1  "MMotorL2Demand"
  Slip Control/2 -> Gain1/1  "MMotorR2Demand"
  Bus Selector/4 -> Slip Control/4  "<gx>"
  Bus Selector/5 -> Slip Control/5  "<gy>"
  Bus Selector/6 -> Slip Control/6  "<nYaw>"

== system sm_car_/Controller/Slip_Ctrl_V2/Spring Damper ==
  Bus Creator : BusCreator  Inputs=4
  Bus Creator1 : BusCreator  Inputs=4
  Constant : Constant  Value=[0 0 0 0]
  Constant1 : Constant  Value=[0 0 0 0]
  Demux : Demux
  Demux1 : Demux
  Damper : Outport  VectorParamsAs1DForOutWhenUnconnected=off
  Spring : Outport  Port=2  VectorParamsAs1DForOutWhenUnconnected=off
  wires:
  Constant/1 -> Demux/1
  Demux/3 -> Bus Creator/3  "L2"
  Demux/4 -> Bus Creator/4  "R2"
  Demux/1 -> Bus Creator/1  "L1"
  Demux/2 -> Bus Creator/2  "R1"
  Demux1/2 -> Bus Creator1/2  "R1"
  Demux1/1 -> Bus Creator1/1  "L1"
  Demux1/4 -> Bus Creator1/4  "R2"
  Demux1/3 -> Bus Creator1/3  "L2"
  Constant1/1 -> Demux1/1
  Bus Creator1/1 -> Damper/1  "Damper"
  Bus Creator/1 -> Spring/1  "Spring"

== system sm_car_/Controller/Slip_Ctrl_V2/Susp ==
  aSteerWheel : Inport
  vx : Inport  Port=2
  1-D Lookup Table : Lookup_n-D  NumberOfTableDimensions=1  BreakpointsForDimension1=Steer.Gain.vVehicle.Value  Table=Steer.Gain.n.Value  InterpMethod=Linear Lagrange  InternalRulePriority=Speed  RndMeth=Simplest
  Bus Creator{1..4} (4 alike) : BusCreator  Inputs=1
  Gain : Gain  Gain=3.6
  Product : Product
  Saturation : Saturate  UpperLimit=Steer.Limits.aUpper.Value  LowerLimit=Steer.Limits.aLower.Value  LinearizeAsGain=off  ZeroCross=off
  Transfer Fcn (with initial states) : simulink_extras/Additional Linear/Transfer Fcn (with initial states)  N=[1]  D="[1/Steer.fActuatorCutoff.Value  1]"  X0=-1
  SuspA1 : Outport  VectorParamsAs1DForOutWhenUnconnected=off
  SuspA2 : Outport  Port=2  VectorParamsAs1DForOutWhenUnconnected=off
  wires:
  Bus Creator4/1 -> Bus Creator1/1  "Steer"
  Bus Creator2/1 -> Bus Creator3/1  "Steer"
  Bus Creator3/1 -> SuspA2/1  "SuspA2"
  Bus Creator1/1 -> SuspA1/1  "SuspA1"
  aSteerWheel/1 -> Product/1, Bus Creator4/1  "aSteerWheel"
  Saturation/1 -> Bus Creator2/1  "aSteerWheel"
  vx/1 -> Gain/1
  Transfer Fcn (with initial states)/1 -> Product/2
  Product/1 -> Saturation/1
  Gain/1 -> 1-D Lookup Table/1
  1-D Lookup Table/1 -> Transfer Fcn (with initial states)/1

== system sm_car_/Controller/TrqVec 4Motor/Brake Control ==
  "rBrakePedal " : Inport
  "VehBus " : Inport  Port=2
  ABS : Subsystem  VariantControl=ABS  mask{abs_tire_radiusF=abs_tire_radiusF, abs_tire_radiusR=abs_tire_radiusR}
      mask prompts: abs_tire_radiusF "Tire Radius Front (m)"; abs_tire_radiusR "Tire Radius Rear (m)"
  Pedal : Subsystem  VariantControl=Pedal
  Pressure : Subsystem  VariantControl=Pressure
  " Brakes" : Outport  VectorParamsAs1DForOutWhenUnconnected=off

== system sm_car_/Controller/TrqVec 4Motor/Driveline Control ==
  Bus Creator : BusCreator  Inputs=1
  Constant : Constant  Value=0
  Driveline : Outport  VectorParamsAs1DForOutWhenUnconnected=off
  wires:
  Bus Creator/1 -> Driveline/1  "Driveline"
  Constant/1 -> Bus Creator/1  "placeholder"

== system sm_car_/Controller/TrqVec 4Motor/Power_TqVec ==
  In Bus Element6 : Inport  PortName=DrvBus  Element=rAccelPedal
  In Bus Element2 : Inport  PortName=DrvBus  Element=aSteerWheel
  In Bus Element3 : Inport  PortName=DrvBus  Element=rBrakePedal
  In Bus Element : Inport  Port=2  PortName=VehBus  Element=Chassis.Body.CG.vx
  In Bus Element1 : Inport  Port=2  PortName=VehBus  Element=Power.MotorL2.w
  In Bus Element8 : Inport  Port=2  PortName=VehBus  Element=Power.MotorR2.w
  In Bus Element5 : Inport  Port=2  PortName=VehBus  Element=World.nYaw
  Bus Creator : BusCreator  Inputs=5
  Constant : Constant  Value=Control.trq_ratio_front
  Constant2 : Constant  Value=1-Control.trq_ratio_front
  Gain1 : Gain  Gain=1600
  Gain3 : Gain  Gain=0.5
  Gain4 : Gain  Gain=0.5
  Product : Product
  Product1 : Product
  Rate Limiter : RateLimiter  RisingSlewLimit=300  FallingSlewLimit=-5000  SampleTimeMode=inherited
  Torque Vectoring : Subsystem  mask(Torque Vectoring, Rear Wheels){vx_enable=Control.vx_enable, aSteerWheel_enable=Control.aSteerWheel_enable, aStr_to_aWhl=Control.aStr_to_aWhl, max_torque_delta=Control.max_torque_delta, P=Control.pGain, I=Control.iGain}
      mask prompts: vx_enable "Speed to enable (m/s)"; aSteerWheel_enable "Steering wheel angle to enable (rad)"; aStr_to_aWhl "Steering Ratio (Wheel/Steering Wheel)"; max_torque_delta "Max Torque Split (N*m)"; P "Simulink:masks:ProportionalP_MP"; I "Simulink:masks:IntegralI_MP"
      mask help: Basic torque vectoring algorithm which applies opposing offsets to the commanded torque of the rear wheels based on the error between the vehicle slip angle and the angle of the steered wheels.
      mask TypeOptions vx_enable: Enable/Enable vx/const
      mask TypeOptions aSteerWheel_enable: Enable/const/Value
      mask TypeOptions aStr_to_aWhl:
      | Vehicle Slip Angle Error/Steering Wheel
      | to Driving Wheel/Gain
      mask TypeOptions max_torque_delta: Max Delta Torque/Value
      mask TypeOptions P: PID Controller/P
      mask TypeOptions I: PID Controller/I
      mask DialogControl P Prompt: Proportional (P):
      mask DialogControl I Prompt: Integral (I):
  Power : Outport  VectorParamsAs1DForOutWhenUnconnected=off
  wires:
  Torque Vectoring/2(trqR2) -> Bus Creator/5  "MMotorR2Demand"
  Torque Vectoring/1(trqL2) -> Bus Creator/4  "MMotorL2Demand"
  In Bus Element3/1 -> Torque Vectoring/7(rBrake)
  In Bus Element5/1 -> Torque Vectoring/6(nYaw)
  In Bus Element8/1 -> Torque Vectoring/5(wR2)
  In Bus Element1/1 -> Torque Vectoring/4(wL2)
  In Bus Element2/1 -> Torque Vectoring/3(aSteerWheel)
  In Bus Element/1 -> Torque Vectoring/2(vx)
  Product1/1 -> Torque Vectoring/1(trqA2)
  Bus Creator/1 -> Power/1  "Power"
  Gain4/1 -> Bus Creator/3  "MMotorR1Demand"
  Gain3/1 -> Bus Creator/2  "MMotorL1Demand"
  Product/1 -> Gain4/1, Gain3/1, Bus Creator/1  "MMotorA1Demand"
  Constant2/1 -> Product1/2
  Constant/1 -> Product/1
  Rate Limiter/1 -> Product/2, Product1/1
  In Bus Element6/1 -> Gain1/1
  Gain1/1 -> Rate Limiter/1

== system sm_car_/Controller/TrqVec 4Motor/Spring Damper ==
  Bus Creator : BusCreator  Inputs=4
  Bus Creator1 : BusCreator  Inputs=4
  Constant : Constant  Value=[0 0 0 0]
  Constant1 : Constant  Value=[0 0 0 0]
  Demux : Demux
  Demux1 : Demux
  Damper : Outport  VectorParamsAs1DForOutWhenUnconnected=off
  Spring : Outport  Port=2  VectorParamsAs1DForOutWhenUnconnected=off
  wires:
  Constant/1 -> Demux/1
  Demux/3 -> Bus Creator/3  "L2"
  Demux/4 -> Bus Creator/4  "R2"
  Demux/1 -> Bus Creator/1  "L1"
  Demux/2 -> Bus Creator/2  "R1"
  Demux1/2 -> Bus Creator1/2  "R1"
  Demux1/1 -> Bus Creator1/1  "L1"
  Demux1/4 -> Bus Creator1/4  "R2"
  Demux1/3 -> Bus Creator1/3  "L2"
  Constant1/1 -> Demux1/1
  Bus Creator1/1 -> Damper/1  "Damper"
  Bus Creator/1 -> Spring/1  "Spring"

== system sm_car_/Controller/TrqVec 4Motor/Susp ==
  aSteerWheel : Inport
  vx : Inport  Port=2
  1-D Lookup Table : Lookup_n-D  NumberOfTableDimensions=1  BreakpointsForDimension1=Steer.Gain.vVehicle.Value  Table=Steer.Gain.n.Value  InterpMethod=Linear Lagrange  InternalRulePriority=Speed  RndMeth=Simplest
  Bus Creator{1..4} (4 alike) : BusCreator  Inputs=1
  Gain : Gain  Gain=3.6
  Product : Product
  Saturation : Saturate  UpperLimit=Steer.Limits.aUpper.Value  LowerLimit=Steer.Limits.aLower.Value  LinearizeAsGain=off  ZeroCross=off
  Transfer Fcn (with initial states) : simulink_extras/Additional Linear/Transfer Fcn (with initial states)  N=[1]  D="[1/Steer.fActuatorCutoff.Value  1]"  X0=-1
  SuspA1 : Outport  VectorParamsAs1DForOutWhenUnconnected=off
  SuspA2 : Outport  Port=2  VectorParamsAs1DForOutWhenUnconnected=off
  wires:
  Bus Creator4/1 -> Bus Creator1/1  "Steer"
  Bus Creator2/1 -> Bus Creator3/1  "Steer"
  Bus Creator3/1 -> SuspA2/1  "SuspA2"
  Bus Creator1/1 -> SuspA1/1  "SuspA1"
  aSteerWheel/1 -> Product/1, Bus Creator4/1  "aSteerWheel"
  Saturation/1 -> Bus Creator2/1  "aSteerWheel"
  vx/1 -> Gain/1
  Transfer Fcn (with initial states)/1 -> Product/2
  Product/1 -> Saturation/1
  Gain/1 -> 1-D Lookup Table/1
  1-D Lookup Table/1 -> Transfer Fcn (with initial states)/1

== system sm_car_/Controller/TrqVec_FLC/Brake Control ==
  "rBrakePedal " : Inport
  "VehBus " : Inport  Port=2
  Pedal : Subsystem  VariantControl=Pedal
  " Brakes" : Outport  VectorParamsAs1DForOutWhenUnconnected=off

== system sm_car_/Controller/TrqVec_FLC/Driveline Control ==
  Bus Creator : BusCreator  Inputs=1
  Constant : Constant  Value=0
  Driveline : Outport  VectorParamsAs1DForOutWhenUnconnected=off
  wires:
  Bus Creator/1 -> Driveline/1  "Driveline"
  Constant/1 -> Bus Creator/1  "placeholder"
